simulink model "BPSK_System_Over_AWGN_Channel"  (R2025b)
settings: Solver=VariableStepAuto  StartTime=0.0  StopTime=inf  RelTol=1e-3
libraries: commchan3 x1, commdigbbndpm3 x1, commrandsrc3 x1, simulink x1, commsink2 x1, commfilt2 x1
settings Model: Creator=Bharath Kumar Reddy  LastModifiedBy=Bharath Kumar Reddy

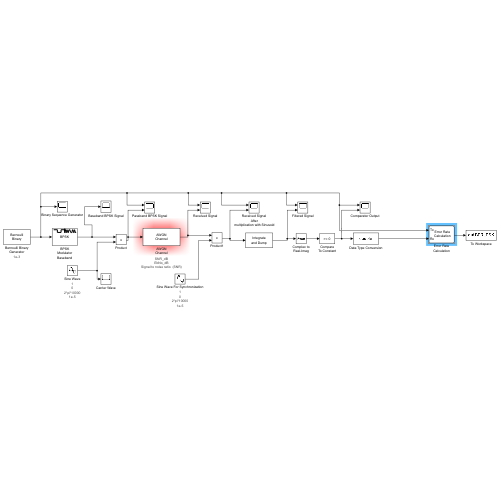
[thumbnail: Simulink's stored preview of the top-level diagram]
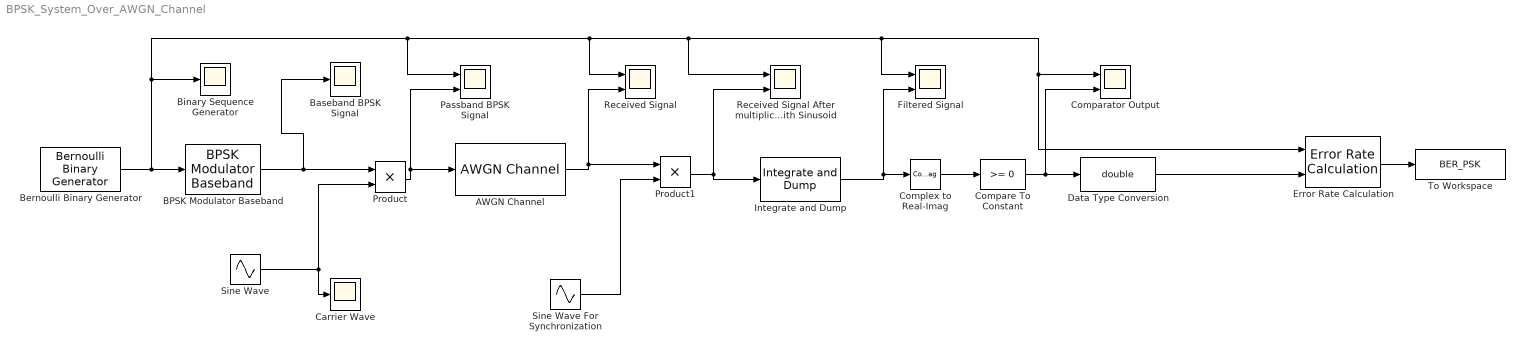
== system BPSK_System_Over_AWGN_Channel ==
  AWGN Channel : commchan3/AWGN Channel  LegacyMode=off  NoiseMethod="Signal to noise ratio  (Eb/No)"  noiseMode="Signal to noise ratio  (SNR)"  EbNo=EbNo_dB  EsNo=10  SNR=SNR_dB  BitsPerSymbol=1  SignalPower=0.5  SpecifySymbolPeriod=off  SamplesPerSymbol=100  SymbolPeriod=1  VarianceSource=Parameter  Variance=1  RandomStream=Global stream  Seed=67  SimulateUsing=Code generation
      settings: AttributesFormatString=|
      | %<SNR>
      | %<EbNo>
      | %<noiseMode>
  BPSK Modulator Baseband : commdigbbndpm3/BPSK Modulator Baseband  Ph=0  outDtype=double  outWordLen=16  outUDDataType=sfix(16)  outFracLenMode=Best precision  outFracLen=15  outDataTypeStr=double  outLastDataTypeStr=double
  Baseband BPSK Signal : Scope
      settings: ActiveDisplayYMinimum=-1.25  ActiveDisplayYMaximum=1.25
  Bernoulli Binary Generator : commrandsrc3/Bernoulli Binary Generator  ProbabilityOfZero=0.5  SeedSource=Auto  Seed=0  SampleTime=1e-3  SamplesPerFrame=1  OutputDataType=double  SimulateUsing=Interpreted execution
      settings: AttributesFormatString=%<SampleTime>
  Binary Sequence Generator : Scope
      settings: ActiveDisplayYMinimum=-1  ActiveDisplayYMaximum=1
  Carrier Wave : Scope
      settings: ActiveDisplayYMinimum=-1  ActiveDisplayYMaximum=1  DataLoggingVariableName=ScopeData5
  Comparator Output : Scope  NumInputPorts=2
      settings: ActiveDisplayYMinimum=-0.12499999999999997  ActiveDisplayYMaximum=1.125  DataLoggingVariableName=ScopeData7
  Compare To Constant : simulink/Logic and Bit Operations/Compare To Constant  relop=>=  const=0  OutDataTypeStr=boolean
  Complex to Real-Imag : ComplexToRealImag  Output=Real
  Data Type Conversion : DataTypeConversion  OutDataTypeStr=double  SaturateOnIntegerOverflow=off  RndMeth=Floor
  Error Rate Calculation : commsink2/Error Rate Calculation  N=1  st_delay=0  cp_mode=Entire frame  subframe=[]  PMode=Port  WsName=ErrorVec  RsMode2=off  stop=on  numErr=100  maxBits=1e4
  Filtered Signal : Scope  NumInputPorts=2
      settings: ActiveDisplayYMinimum=-1.1792984362590477  ActiveDisplayYMaximum=1.2421442706954497  DataLoggingVariableName=ScopeData6
  Integrate and Dump : commfilt2/Integrate and Dump  obssamples=100  offsetsamples=0  nodump=off  roundingMode=Floor  overflowMode=off  outputDataTypeStr=Inherit: Same as accumulator  outputLastDataTypeStr=Inherit: Same as accumulator
  Passband BPSK Signal : Scope  NumInputPorts=2
      settings: ActiveDisplayYMinimum=-1.2500000000000009  ActiveDisplayYMaximum=1.2500000000000007  DataLoggingVariableName=ScopeData2
  Product : Product
  Product1 : Product
  Received Signal : Scope  NumInputPorts=2
      settings: ActiveDisplayYMinimum=-1.1891290394577225  ActiveDisplayYMaximum=1.1891185308089534  DataLoggingVariableName=ScopeData3
  Received Signal After multiplication with Sinusoid : Scope  NumInputPorts=2
      settings: ActiveDisplayYMinimum=-1  ActiveDisplayYMaximum=1  DataLoggingVariableName=ScopeData4
  Sine Wave : Sin  Frequency=2*pi*10000  SampleTime=1e-5
      settings: AttributesFormatString=|
      | %<Amplitude>
      | %<Bias>
      | %<Frequency>
      | %<SampleTime>
  Sine Wave For Synchronization : Sin  Frequency=2*pi*10000  Phase=pi  SampleTime=1e-5
      settings: AttributesFormatString=|
      | %<Amplitude>
      | %<Bias>
      | %<Frequency>
      | %<SampleTime>
  To Workspace : ToWorkspace  VariableName=BER_PSK  SaveFormat=Timeseries  SampleTime=-1
  wires:
  BPSK Modulator Baseband/1 -> Baseband BPSK Signal/1, Product/1
  Sine Wave/1 -> Carrier Wave/1, Product/2
  Product/1 -> Passband BPSK Signal/2, AWGN Channel/1
  Bernoulli Binary Generator/1 -> Received Signal/1, Error Rate Calculation/1, Comparator Output/1, Filtered Signal/1, Received Signal After multiplication with Sinusoid/1, Passband BPSK Signal/1, Binary Sequence Generator/1, BPSK Modulator Baseband/1
  AWGN Channel/1 -> Product1/1, Received Signal/2
  Product1/1 -> Integrate and Dump/1, Received Signal After multiplication with Sinusoid/2
  Sine Wave For Synchronization/1 -> Product1/2
  Integrate and Dump/1 -> Complex to Real-Imag/1, Filtered Signal/2
  Complex to Real-Imag/1 -> Compare To Constant/1
  Compare To Constant/1 -> Data Type Conversion/1, Comparator Output/2
  Data Type Conversion/1 -> Error Rate Calculation/2
  Error Rate Calculation/1 -> To Workspace/1
